simulink model "BMS"  (R2024a)
settings: Solver=VariableStepAuto  StartTime=0.0  StopTime=300  RelTol=1e-3
libraries: fl_lib x7, nesl_utility x2, batteryecm_lib x1, ee_lib x1
settings Model: Creator=liubo  LastModifiedBy=liubo

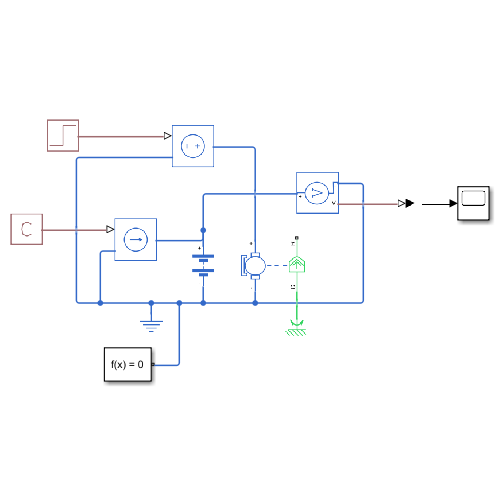
[thumbnail: Simulink's stored preview of the top-level diagram]
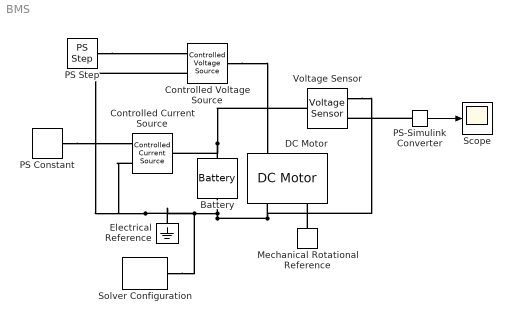
== system BMS ==
  Battery : batteryecm_lib/Battery  Vnom=3.7 V  prm_dir=simscape.enum.battery.prm_dir.disabled  R1_dis=2 Ohm  R1_ch=2 Ohm  R1=5 mOhm  prm_AH=simscape.enum.battery.prm_AH.finite  AH=500 mAh  V1=3.6 V  AH1=250 mAh  prm_R2=simscape.enum.battery.prm_R2.disabled  R2=2000 Ohm  Tmeas=298.15 K  charge_measurement_port=simscape.enum.battery.enable.no  prm_dyn=simscape.enum.battery.prm_dyn.off  Rp1=0.005 Ohm  tau1=30 s  Rp2=0.005 Ohm  tau2=30 s  Rp3=0.005 Ohm  tau3=30 s  Rp4=0.005 Ohm  tau4=30 s  Rp5=0.005 Ohm  tau5=30 s  prm_fade=simscape.enum.battery.prm_fade.disabled  N_fade=100  AH_fade=45 A*hr  R1_fade=2.02 Ohm  R1_ch_fade=2.02 Ohm  V1_fade=10.35 V  prm_age=simscape.enum.battery.prm_age.disabled  prm_age_OCV=simscape.enum.battery.prm_age_OCV.OCV  OCV_age=0.9  SOC_age=60  Tmeas_age=298.15 K  delta_time_age_vec=[0] d  temperature_age_vec=[273] K  OCV_scaling_age=2.2134e6  OCV_offset_age=1.632e6  temp_exp_age=0.515833569 V  t_exp_age=0.75  Vnom_T2=12 V  R1_T2=2.2 Ohm  R1_T2_dis=2.2 Ohm  R1_T2_ch=2.2 Ohm  V1_T2=11.4 V  R2_T2=2200 Ohm  Rp1_T2=0.005 Ohm  tau1_T2=30 s  Rp2_T2=0.005 Ohm  tau2_T2=30 s  Rp3_T2=0.005 Ohm  tau3_T2=30 s  Rp4_T2=0.005 Ohm  tau4_T2=30 s  Rp5_T2=0.005 Ohm  tau5_T2=30 s  Tmeas2=273.15 K  thermal_port=simscape.enum.thermaleffects.omit  thermal_mass=30000 J/K  i_specify=off  i_priority=None  i=0 A  i_nominal_specify=off  i_nominal_value=1  i_nominal_unit=A  v_specify=off  v_priority=None  v=0 V  v_nominal_specify=off  v_nominal_value=1  v_nominal_unit=V  charge_specify=off  charge_priority=High  charge=50 A*hr  charge_nominal_specify=off  charge_nominal_value=1  charge_nominal_unit=A*hr  num_cycles_specify=off  num_cycles_priority=High  num_cycles=0  num_cycles_nominal_specify=off  num_cycles_nominal_value=1  num_cycles_nominal_unit=1  temperature_specify=off  temperature_priority=High  temperature=298.15 K  temperature_nominal_specify=off  temperature_nominal_value=1  temperature_nominal_unit=K
  Controlled Current Source : fl_lib/Electrical/Electrical Sources/Controlled Current Source
  Controlled Voltage Source : fl_lib/Electrical/Electrical Sources/Controlled Voltage Source
  DC Motor : ee_lib/Electromechanical/Brushed Motors/DC Motor  field_option=ee.enum.field_option.pm  Rf=100 Ohm  Lf=1 H  Laf=0.15 H  If0=0 A  parameterization=ee.enum.dcparam_option.circuit_param  Ra=12 Ohm  La=1 mH  emf_or_torque=ee.enum.emf_or_torque.kv  Kv=1.1e-3 V/rpm  Ki=6.876e-4 N*m/A  T_stall=0.24e-3 N*m  w_max=19100 rpm  w_rated=15000 rpm  P_rated=0.08 W  V_rated=1.5 V  lam_param=ee.enum.lam_param.damping  i_noload=0 A  V_i_noload=1.5 V  J=0.01 cm^2*g  lam=0 N*m*s/rad  speed0=0 rpm  enable_fault_armature=simscape.enum.onoff.off  rev_faulted=1 / 3  G_faulted_armature=1e-5 S  fault_trigger_armature=ee.enum.faults.faultTrigger.temporal  t_fault_armature=1 s  max_permissible_current_armature=inf A  t_fail_on_current_armature=1 s  enable_fault_field=simscape.enum.onoff.off  G_faulted_field=1e-5 S  fault_trigger_field=ee.enum.faults.faultTrigger.temporal  t_fault_field=1 s  max_permissible_current_field=inf A  t_fail_on_current_field=1 s  fault_action=simscape.enum.assert.action.none  alpha=3.93e-3 1/K  Tmeas=25 degC  thermal_mass=100 J/K  initial_temperature=25 degC
  Electrical Reference : fl_lib/Electrical/Electrical Elements/Electrical Reference
  Mechanical Rotational Reference : fl_lib/Mechanical/Rotational Elements/Mechanical Rotational Reference
  PS Constant : fl_lib/Physical Signals/Sources/PS Constant  constant=0.06 A
  PS Step : fl_lib/Physical Signals/Sources/PS Step  step_time=5 s  initial_value=0  final_value=3.7
  PS-Simulink Converter : nesl_utility/PS-Simulink Converter  PhysicalDomain=network_engine_domain  SubClassName=ps_output  LeftPortType=input  RightPortType=output  PseudoPeriodic=off  Frequencies=[]  VectorFormat=inherit  Unit=inherit  AffineConversion=off
  Scope : Scope
  Solver Configuration : nesl_utility/Solver Configuration  PhysicalDomain=network_engine_domain  SubClassName=solver  LeftPortType=input  RightPortType=generic  Tones=[]  Harmonics=[]  SimulateNoise=off  Profile=off  UseLocalSampling=off  EnableSwitchedLinearOptims=on  FrequencyDomain=off  UseCCode=off  RelTol=0.001  AbsTol=0.001  MinStep=1e-09  ToWorkspace=off  RevertToSquareIcSolve=off  NumHomotopyIterations=100  PhasorMode=off  PhasorModeNumHarmonics=1  ConsistencySolver=NEWTON_XTOL_AFTER_FTOL  IndexReductionMethod=DerivativeReplacement  DoDC=off  ResidualTolerance=1e-09  ConsistencyTolSource=GLOBAL  ConsistencyAbsTol=0.001  ConsistencyRelTol=0.001  ConsistencyTolFactor=0.001  UseLocalSolver=off  LocalSolverChoice=NE_BACKWARD_EULER_ADVANCER  ResolveIndetEquations=on  FunctionEvalNumThread=1  LocalSolverSampleTime=0.001  DoFixedCost=off  MaxNonlinIter=3  MaxModeIter=2  ComputeImpulses=off  ImpulseIterations=2  LinearAlgebra=auto  LinearAlgebraNumThread=0  EquationFormulation=NE_TIME_EF  DelaysMemoryBudget=1024  AutomaticFiltering=on  FilteringTimeConstant=0.001  PartitionStorageMethod=AS_NEEDED  PartitionMemoryBudget=1024  PartitionMethod=ROBUST  MultibodyUseLocalSolver=off  MultibodyLocalSolverChoice=ODE1  MultibodyLocalSolverSampleTime=0.001
  Voltage Sensor : fl_lib/Electrical/Electrical Sensors/Voltage Sensor
  wires:
  PS-Simulink Converter/1 -> Scope/1
  connections:
  PS Constant/RConn1 -- Controlled Current Source/RConn1
  Battery/LConn1 -- Voltage Sensor/LConn1 -- Controlled Current Source/LConn1
  DC Motor/RConn1 -- Solver Configuration/RConn1 -- Controlled Voltage Source/RConn2 -- Controlled Current Source/RConn2 -- Electrical Reference/LConn1 -- Battery/RConn1 -- Voltage Sensor/RConn2
  PS Step/RConn1 -- Controlled Voltage Source/RConn1
  Controlled Voltage Source/LConn1 -- DC Motor/LConn1
  PS-Simulink Converter/LConn1 -- Voltage Sensor/RConn1
  Mechanical Rotational Reference/LConn1 -- DC Motor/RConn2
